simulink model "V5_Current_Field_Loop"  (R2025b)
settings: Solver=FixedStepDiscrete  StartTime=0.0  StopTime=119.4005  FixedStep=.0005  RelTol=1e-3
libraries: modelsimlib x1
settings Model: Creator=李晨光  LastModifiedBy=李晨光
settings DataIOCC: SignalLogging=off
settings DebuggingCC: AlgebraicLoopMsg=error

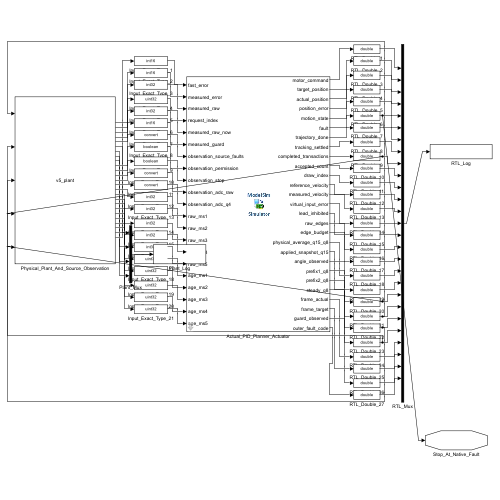
[thumbnail: Simulink's stored preview of the top-level diagram]
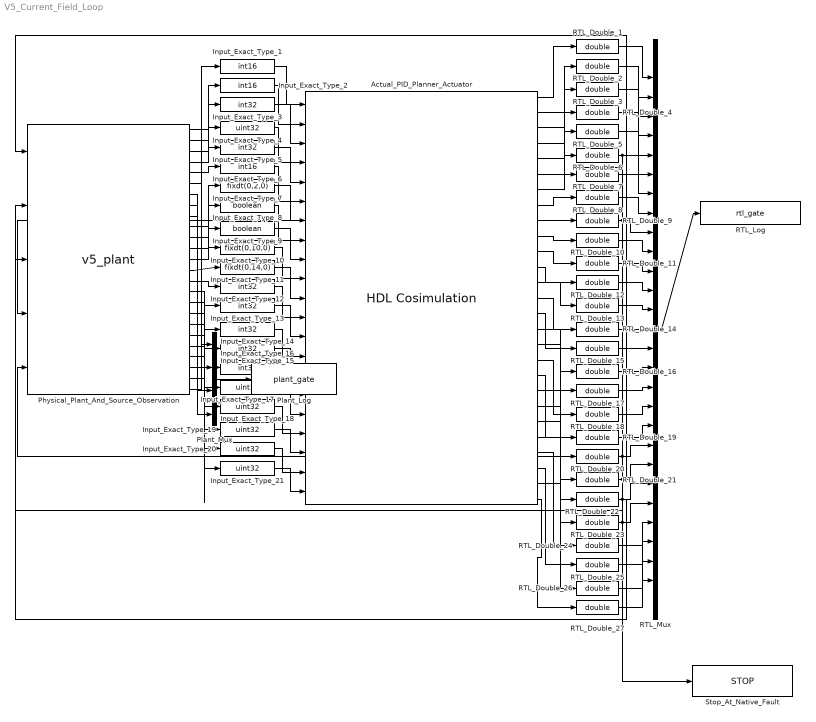
== system V5_Current_Field_Loop ==
  Actual_PID_Planner_Actuator : modelsimlib/HDL Cosimulation  PortPaths=/v5_cosim_core/fast_error;/v5_cosim_core/measured_error;/v5_cosim_core/measured_raw;/v5_cosim_core/request_index;/v5_cosim_core/measured_raw_now;/v5_cosim_core/measured_guard;/v5_cosim_core/observation_source_faults;/v5_cosim_core/observation_permission;/v5_cosim_core/observation_stop;/v5_cosim_core/observation_adc_raw;/v5_cosim_core/observation_adc_q4;/v5_cosim_core/raw_ms1;/v5_cosim_core/raw_ms2;/v5_cosim_core/raw_ms3;/v5_cosim_core/raw_ms4;/v5_cosim_core/raw_ms5;/v5_cosim_core/age_ms1;/v5_cosim_core/age_ms2;/v5_cosim_core/age_ms3;/v5_cosim_core/age_ms4;/v5_cosim_core/age_ms5;/v5_cosim_core/motor_command;/v5_cosim_core/target_position;/v5_cosim_core/actual_position;/v5_cosim_core/position_error;/v5_cosim_core/motion_state;/v5_cosim_core/fault;/v5_cosim_core/trajectory_done;/v5_cosim_core/tracking_settled;/v5_cosim_core/completed_transactions;/v5_cosim_core/accepted_count;/v5_cosim_core/draw_index;/v5_cosim_core/reference_velocity;/v5_cosim_core/measured_velocity;/v5_cosim_core/virtual_input_error;/v5_cosim_core/lead_inhibited;/v5_cosim_core/raw_edges;/v5_cosim_core/edge_budget;/v5_cosim_core/physical_average_q15_q8;/v5_cosim_core/applied_snapshot_q15;/v5_cosim_core/angle_observed;/v5_cosim_core/prefix1_q8;/v5_cosim_core/prefix2_q8;/v5_cosim_core/steady_q8;/v5_cosim_core/frame_actual;/v5_cosim_core/frame_target;/v5_cosim_core/guard_observed;/v5_cosim_core/outer_fault_code  PortModes=[1 1 1 1 1 1 1 1 1 1 1 1 1 1 1 1 1 1 1 1 1 2 2 2 2 2 2 2 2 2 2 2 2 2 2 2 2 2 2 2 2 2 2 2 2 2 2 2]  PortTimes=[-1 -1 -1 -1 -1 -1 -1 -1 -1 -1 -1 -1 -1 -1 -1 -1 -1 -1 -1 -1 -1 0.0005 0.0005 0.0005 0.0005 0.0005 0.0005 0.0005 0.0005 0.0005 0.0005 0.0005 0.0005 0.0005 0.0005 0.0005 0.0005 0.0005 0.0005 0.0005 0.0005 0.0005 0.0005 0.0005 0.0005 0.0005 0.0005 0.0005]  PortSigns=[-1 -1 -1 -1 -1 -1 -1 -1 -1 -1 -1 -1 -1 -1 -1 -1 -1 -1 -1 -1 -1 1 1 1 1 0 0 0 0 0 0 0 1 1 1 1 1 1 1 1 1 1 1 1 1 1 1 0]  PortFracLengths=[0 0 0 0 0 0 0 0 0 0 0 0 0 0 0 0 0 0 0 0 0 0 0 0 0 0 0 0 0 0 0 0 0 0 0 0 0 0 0 0 0 0 0 0 0 0 0 0]  PortWordLengths=[-1 -1 -1 -1 -1 -1 -1 -1 -1 -1 -1 -1 -1 -1 -1 -1 -1 -1 -1 -1 -1 -1 -1 -1 -1 -1 -1 -1 -1 -1 -1 -1 -1 -1 -1 -1 -1 -1 -1 -1 -1 -1 -1 -1 -1 -1 -1 -1]  PortHDLWordSizes=[0 0 0 0 0 0 0 0 0 0 0 0 0 0 0 0 0 0 0 0 0 0 0 0 0 0 0 0 0 0 0 0 0 0 0 0 0 0 0 0 0 0 0 0 0 0 0 0]  CommLocal=on  CommSharedMemory=off  CommPortNumber=4869  CommShowInfo=off  ClockModes=[]  ClockTimes=[]  TclPreSimCommand=puts {V5_CURRENT_FIELD_BEGIN}  TclPostSimCommand=puts {V5_CURRENT_FIELD_END}  TimingMode=Tick  TimingScaleFactor=1e9  idxCellArray={'UNUSED_VAR'}  CosimBypass=Full Simulation  AllowDirectFeedthrough=on  ProductName=EDA Simulator Link MQ  RunAutoTimescale=off  HdlClocks=0  PreRunTime=3  PreRunTimeUnit=ms
  Input_Exact_Type_1 : DataTypeConversion  OutDataTypeStr=int16  SaturateOnIntegerOverflow=off  RndMeth=Floor
  Input_Exact_Type_10 : DataTypeConversion  OutDataTypeStr=fixdt(0,10,0)  SaturateOnIntegerOverflow=off  RndMeth=Floor
  Input_Exact_Type_11 : DataTypeConversion  OutDataTypeStr=fixdt(0,14,0)  SaturateOnIntegerOverflow=off  RndMeth=Floor
  Input_Exact_Type_{3,5,12..16} (7 alike) : DataTypeConversion  OutDataTypeStr=int32  SaturateOnIntegerOverflow=off  RndMeth=Floor
  Input_Exact_Type_{4,17..21} (6 alike) : DataTypeConversion  OutDataTypeStr=uint32  SaturateOnIntegerOverflow=off  RndMeth=Floor
  Input_Exact_Type_2 : DataTypeConversion  OutDataTypeStr=int16  SaturateOnIntegerOverflow=off  RndMeth=Floor
  Input_Exact_Type_6 : DataTypeConversion  OutDataTypeStr=int16  SaturateOnIntegerOverflow=off  RndMeth=Floor
  Input_Exact_Type_7 : DataTypeConversion  OutDataTypeStr=fixdt(0,2,0)  SaturateOnIntegerOverflow=off  RndMeth=Floor
  Input_Exact_Type_8 : DataTypeConversion  OutDataTypeStr=boolean  SaturateOnIntegerOverflow=off  RndMeth=Floor
  Input_Exact_Type_9 : DataTypeConversion  OutDataTypeStr=boolean  SaturateOnIntegerOverflow=off  RndMeth=Floor
  Physical_Plant_And_Source_Observation : M-S-Function  FunctionName=v5_plant
  Plant_Log : ToWorkspace  VariableName=plant_gate  SaveFormat=Timeseries  SampleTime=-1
  Plant_Mux : Mux
  RTL_Double_{1..27} (27 alike) : DataTypeConversion  OutDataTypeStr=double  SaturateOnIntegerOverflow=off  RndMeth=Floor
  RTL_Log : ToWorkspace  VariableName=rtl_gate  SaveFormat=Timeseries  SampleTime=-1
  RTL_Mux : Mux  Inputs=27
  Stop_At_Native_Fault : Stop
  wires:
  Physical_Plant_And_Source_Observation/25 -> Input_Exact_Type_1/1
  Input_Exact_Type_1/1 -> Actual_PID_Planner_Actuator/1
  Physical_Plant_And_Source_Observation/1 -> Input_Exact_Type_2/1
  Input_Exact_Type_2/1 -> Actual_PID_Planner_Actuator/2
  Physical_Plant_And_Source_Observation/2 -> Input_Exact_Type_3/1
  Input_Exact_Type_3/1 -> Actual_PID_Planner_Actuator/3
  Physical_Plant_And_Source_Observation/3 -> Input_Exact_Type_4/1
  Input_Exact_Type_4/1 -> Actual_PID_Planner_Actuator/4
  Physical_Plant_And_Source_Observation/4 -> Input_Exact_Type_5/1
  Input_Exact_Type_5/1 -> Actual_PID_Planner_Actuator/5
  Physical_Plant_And_Source_Observation/5 -> Input_Exact_Type_6/1
  Input_Exact_Type_6/1 -> Actual_PID_Planner_Actuator/6
  Physical_Plant_And_Source_Observation/10 -> Input_Exact_Type_7/1
  Input_Exact_Type_7/1 -> Actual_PID_Planner_Actuator/7
  Physical_Plant_And_Source_Observation/11 -> Input_Exact_Type_8/1
  Input_Exact_Type_8/1 -> Actual_PID_Planner_Actuator/8
  Physical_Plant_And_Source_Observation/12 -> Input_Exact_Type_9/1
  Input_Exact_Type_9/1 -> Actual_PID_Planner_Actuator/9
  Physical_Plant_And_Source_Observation/13 -> Input_Exact_Type_10/1
  Input_Exact_Type_10/1 -> Actual_PID_Planner_Actuator/10
  Physical_Plant_And_Source_Observation/14 -> Input_Exact_Type_11/1
  Input_Exact_Type_11/1 -> Actual_PID_Planner_Actuator/11
  Physical_Plant_And_Source_Observation/15 -> Input_Exact_Type_12/1
  Input_Exact_Type_12/1 -> Actual_PID_Planner_Actuator/12
  Physical_Plant_And_Source_Observation/16 -> Input_Exact_Type_13/1
  Input_Exact_Type_13/1 -> Actual_PID_Planner_Actuator/13
  Physical_Plant_And_Source_Observation/17 -> Input_Exact_Type_14/1
  Input_Exact_Type_14/1 -> Actual_PID_Planner_Actuator/14
  Physical_Plant_And_Source_Observation/18 -> Input_Exact_Type_15/1
  Input_Exact_Type_15/1 -> Actual_PID_Planner_Actuator/15
  Physical_Plant_And_Source_Observation/19 -> Input_Exact_Type_16/1
  Input_Exact_Type_16/1 -> Actual_PID_Planner_Actuator/16
  Physical_Plant_And_Source_Observation/20 -> Input_Exact_Type_17/1
  Input_Exact_Type_17/1 -> Actual_PID_Planner_Actuator/17
  Physical_Plant_And_Source_Observation/21 -> Input_Exact_Type_18/1
  Input_Exact_Type_18/1 -> Actual_PID_Planner_Actuator/18
  Physical_Plant_And_Source_Observation/22 -> Input_Exact_Type_19/1
  Input_Exact_Type_19/1 -> Actual_PID_Planner_Actuator/19
  Physical_Plant_And_Source_Observation/23 -> Input_Exact_Type_20/1
  Input_Exact_Type_20/1 -> Actual_PID_Planner_Actuator/20
  Physical_Plant_And_Source_Observation/24 -> Input_Exact_Type_21/1
  Input_Exact_Type_21/1 -> Actual_PID_Planner_Actuator/21
  Actual_PID_Planner_Actuator/1 -> RTL_Double_1/1
  Actual_PID_Planner_Actuator/2 -> RTL_Double_2/1
  Actual_PID_Planner_Actuator/3 -> RTL_Double_3/1
  Actual_PID_Planner_Actuator/4 -> RTL_Double_4/1
  Actual_PID_Planner_Actuator/5 -> RTL_Double_5/1
  Actual_PID_Planner_Actuator/6 -> RTL_Double_6/1
  Actual_PID_Planner_Actuator/7 -> RTL_Double_7/1
  Actual_PID_Planner_Actuator/8 -> RTL_Double_8/1
  Actual_PID_Planner_Actuator/9 -> RTL_Double_9/1
  Actual_PID_Planner_Actuator/10 -> RTL_Double_10/1
  Actual_PID_Planner_Actuator/11 -> RTL_Double_11/1
  Actual_PID_Planner_Actuator/12 -> RTL_Double_12/1
  Actual_PID_Planner_Actuator/13 -> RTL_Double_13/1
  Actual_PID_Planner_Actuator/14 -> RTL_Double_14/1
  Actual_PID_Planner_Actuator/15 -> RTL_Double_15/1
  Actual_PID_Planner_Actuator/16 -> RTL_Double_16/1
  Actual_PID_Planner_Actuator/17 -> RTL_Double_17/1
  Actual_PID_Planner_Actuator/18 -> RTL_Double_18/1
  Actual_PID_Planner_Actuator/19 -> RTL_Double_19/1
  Actual_PID_Planner_Actuator/20 -> RTL_Double_20/1
  Actual_PID_Planner_Actuator/21 -> RTL_Double_21/1
  Actual_PID_Planner_Actuator/22 -> RTL_Double_22/1
  Actual_PID_Planner_Actuator/23 -> RTL_Double_23/1
  Actual_PID_Planner_Actuator/24 -> RTL_Double_24/1
  Actual_PID_Planner_Actuator/25 -> RTL_Double_25/1
  Actual_PID_Planner_Actuator/26 -> RTL_Double_26/1
  Actual_PID_Planner_Actuator/27 -> RTL_Double_27/1
  RTL_Double_21/1 -> Physical_Plant_And_Source_Observation/1, RTL_Mux/21
  RTL_Double_22/1 -> Physical_Plant_And_Source_Observation/2, RTL_Mux/22
  RTL_Double_23/1 -> Physical_Plant_And_Source_Observation/3, RTL_Mux/23
  RTL_Double_9/1 -> Physical_Plant_And_Source_Observation/4, RTL_Mux/9
  RTL_Double_20/1 -> Physical_Plant_And_Source_Observation/5, RTL_Mux/20
  RTL_Double_1/1 -> RTL_Mux/1
  RTL_Double_2/1 -> RTL_Mux/2
  RTL_Double_3/1 -> RTL_Mux/3
  RTL_Double_4/1 -> RTL_Mux/4
  RTL_Double_5/1 -> RTL_Mux/5
  RTL_Double_6/1 -> RTL_Mux/6, Stop_At_Native_Fault/1
  RTL_Double_7/1 -> RTL_Mux/7
  RTL_Double_8/1 -> RTL_Mux/8
  RTL_Double_10/1 -> RTL_Mux/10
  RTL_Double_11/1 -> RTL_Mux/11
  RTL_Double_12/1 -> RTL_Mux/12
  RTL_Double_13/1 -> RTL_Mux/13
  RTL_Double_14/1 -> RTL_Mux/14
  RTL_Double_15/1 -> RTL_Mux/15
  RTL_Double_16/1 -> RTL_Mux/16
  RTL_Double_17/1 -> RTL_Mux/17
  RTL_Double_18/1 -> RTL_Mux/18
  RTL_Double_19/1 -> RTL_Mux/19
  RTL_Double_24/1 -> RTL_Mux/24
  RTL_Double_25/1 -> RTL_Mux/25
  RTL_Double_26/1 -> RTL_Mux/26
  RTL_Double_27/1 -> RTL_Mux/27
  RTL_Mux/1 -> RTL_Log/1
  Physical_Plant_And_Source_Observation/6 -> Plant_Mux/1
  Physical_Plant_And_Source_Observation/7 -> Plant_Mux/2
  Physical_Plant_And_Source_Observation/8 -> Plant_Mux/3
  Physical_Plant_And_Source_Observation/9 -> Plant_Mux/4
  Plant_Mux/1 -> Plant_Log/1
